simulink model "dc_motor_speed_control"  (R2025b)
settings: Solver=ode45  StartTime=0.0  StopTime=p.stopTime  MaxStep=0.002  RelTol=1e-8  AbsTol=1e-10
model workspace (MAT data in the model file):
  p.R = 1.2
  p.L = 0.02
  p.J = 0.004
  p.b = 0.002
  p.Kt = 0.08
  p.Ke = 0.08
  p.Kp = 0.4
  p.Ki = 4
  p.Kd = 0.002
  p.N = 150
  p.Kaw = 20
  p.voltageLimit = 24
  p.reference = 120
  p.referenceTime = 0.1
  p.loadTorque = 0.12
  p.loadTime = 2.508
  p.stopTime = 3.734
  p.sampleTime = 0.002
settings Model: Creator=LENOVO  LastModifiedBy=LENOVO

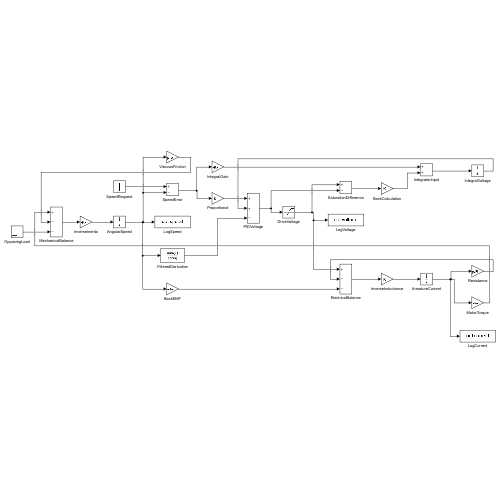
[thumbnail: Simulink's stored preview of the top-level diagram]
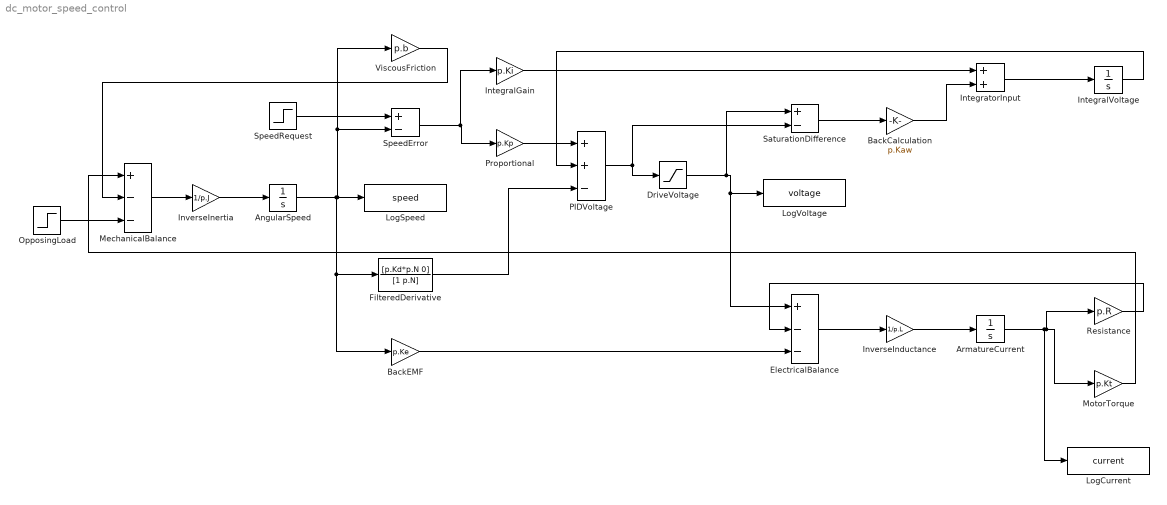
== system dc_motor_speed_control ==
  AngularSpeed : Integrator
  ArmatureCurrent : Integrator
  BackCalculation : Gain  Gain=p.Kaw
  BackEMF : Gain  Gain=p.Ke
  DriveVoltage : Saturate  UpperLimit=p.voltageLimit  LowerLimit=-p.voltageLimit
  ElectricalBalance : Sum  Inputs=+--
  FilteredDerivative : TransferFcn  Numerator=[p.Kd*p.N 0]  Denominator=[1 p.N]
  IntegralGain : Gain  Gain=p.Ki
  IntegralVoltage : Integrator
  IntegratorInput : Sum
  InverseInductance : Gain  Gain=1/p.L
  InverseInertia : Gain  Gain=1/p.J
  LogCurrent : ToWorkspace  VariableName=current  SaveFormat=Timeseries  SampleTime=-1
  LogSpeed : ToWorkspace  VariableName=speed  SaveFormat=Timeseries  SampleTime=-1
  LogVoltage : ToWorkspace  VariableName=voltage  SaveFormat=Timeseries  SampleTime=-1
  MechanicalBalance : Sum  Inputs=+--
  MotorTorque : Gain  Gain=p.Kt
  OpposingLoad : Step  Time=p.loadTime  After=p.loadTorque  SampleTime=0
  PIDVoltage : Sum  Inputs=++-
  Proportional : Gain  Gain=p.Kp
  Resistance : Gain  Gain=p.R
  SaturationDifference : Sum  Inputs=+-
  SpeedError : Sum  Inputs=+-
  SpeedRequest : Step  Time=p.referenceTime  After=p.reference  SampleTime=0
  ViscousFriction : Gain  Gain=p.b
  wires:
  InverseInertia/1 -> AngularSpeed/1
  MechanicalBalance/1 -> InverseInertia/1
  OpposingLoad/1 -> MechanicalBalance/3
  ViscousFriction/1 -> MechanicalBalance/2
  MotorTorque/1 -> MechanicalBalance/1
  ArmatureCurrent/1 -> Resistance/1, MotorTorque/1, LogCurrent/1
  InverseInductance/1 -> ArmatureCurrent/1
  ElectricalBalance/1 -> InverseInductance/1
  BackEMF/1 -> ElectricalBalance/3
  Resistance/1 -> ElectricalBalance/2
  SaturationDifference/1 -> BackCalculation/1
  DriveVoltage/1 -> ElectricalBalance/1, LogVoltage/1, SaturationDifference/1
  PIDVoltage/1 -> DriveVoltage/1, SaturationDifference/2
  FilteredDerivative/1 -> PIDVoltage/3
  IntegralVoltage/1 -> PIDVoltage/2
  Proportional/1 -> PIDVoltage/1
  IntegratorInput/1 -> IntegralVoltage/1
  BackCalculation/1 -> IntegratorInput/2
  IntegralGain/1 -> IntegratorInput/1
  SpeedError/1 -> Proportional/1, IntegralGain/1
  AngularSpeed/1 -> BackEMF/1, FilteredDerivative/1, ViscousFriction/1, SpeedError/2, LogSpeed/1
  SpeedRequest/1 -> SpeedError/1
